simulink model "S5_MPC_Lab"  (R2025b)
settings: Solver=VariableStepAuto  StartTime=0.0  StopTime=200  FixedStep=0.5  MaxStep=0.05  RelTol=1e-3  AbsTol=1e-3
undefined symbols (not defined in the file or in its folder): g, gamma, mpc_Ts, q_in_step, T_water
libraries: nesl_utility x5, SimscapeFluids_lib x5, fl_lib x3, mpclib x1
settings Model: PacingRate=3.966100  Creator=emanu  LastModifiedBy=leffe
settings SolverCC: AutoScaleAbsTol=off  AlgebraicLoopSolver=TrustRegion  MaxZcPerStep=1.0
settings OptimizationCC: ReuseModelBlockBuffer=off
settings DebuggingCC: AlgebraicLoopMsg=none  UnconnectedInputMsg=warning  UnconnectedOutputMsg=warning  UnconnectedLineMsg=warning  SymbolicDimsDataTypeCodeGenerationDiagnostic=none
settings ModelReferenceCC: EnableRefExpFcnMdlSchedulingChecks=on
settings SFSimCC: CustomCodeUndefinedFunction=UseInterfaceOnly
settings RTWCC: GPUComputeCapability=3.5  DLArmComputeVersion=19.05
settings SimscapeCC: SimscapeLogDataHistory=10000.0

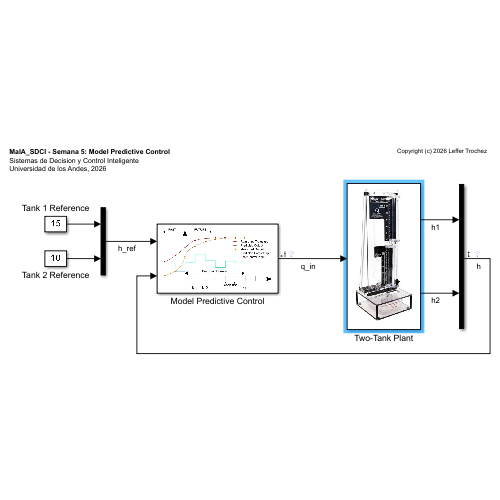
[thumbnail: Simulink's stored preview of the top-level diagram]
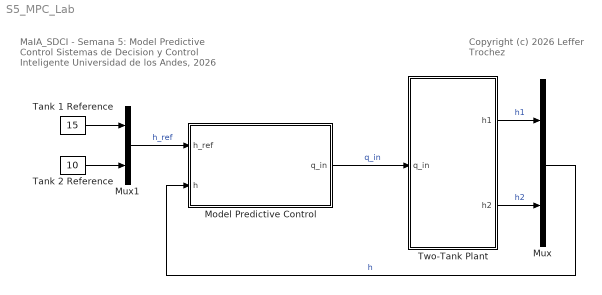
== system S5_MPC_Lab ==
  note: MaIA_SDCI - Semana 5: Model Predictive Control
      | Sistemas de Decision y Control Inteligente
      | Universidad de los Andes, 2026
  note: Copyright (c) 2026 Leffer Trochez
  Model Predictive Control : Subsystem
      mask Display: image('MPC.webp', [0,0,0,0,90,90]);
  Mux : Mux  Inputs=2
  Mux1 : Mux  Inputs=2
  Tank 1 Reference : Constant  Value=15
  Tank 2 Reference : Constant  Value=10
  Two-Tank Plant : Subsystem
      mask Display: image('Plant.jpeg');
  wires:
  Model Predictive Control/1(q_in) -> Two-Tank Plant/1(q_in)  "q_in"
  Two-Tank Plant/1(h1) -> Mux/1  "h1"
  Two-Tank Plant/2(h2) -> Mux/2  "h2"
  Mux/1 -> Model Predictive Control/2(h)  "h"
  Mux1/1 -> Model Predictive Control/1(h_ref)  "h_ref"
  Tank 1 Reference/1 -> Mux1/1
  Tank 2 Reference/1 -> Mux1/2

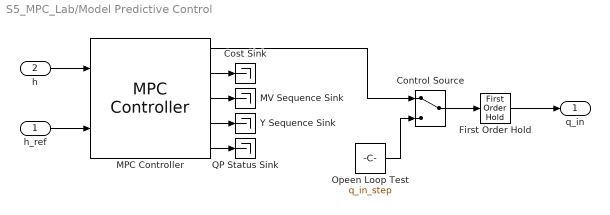
== system S5_MPC_Lab/Model Predictive Control ==
  h_ref : Inport
  h : Inport  Port=2
  " First Order Hold " : FirstOrderHold  ErrorTolerance=inf
  " MPC Controller " : mpclib/MPC Controller  SCDEnableBlockLinearizationSpecification=on  mpcobj=mpcController  is_multiple=0  enable_value=0  return_u0=off  updateMPCinCallerWorkspace=on  md_inport=off  mv_inport=off  uref_inport=off  return_cost=on  return_mvseq=on  return_qpstatus=on  return_xseq=off  return_state=off  return_ovseq=on  state_inport=off  umin_inport=off  umax_inport=off  ymin_inport=off  ymax_inport=off  cc_inport=off  ywt_inport=off  uwt_inport=off  duwt_inport=off  rhoeps_inport=off  pm_inport=off  MaximumP=10  HorizonChoice=FixedHorizon  n_ts=0.5  n_p=40  n_mv=1  n_md=0  n_ud=0  n_mo=2  n_uo=0  BlockDataType=double  SampleTimeInherited=off  switch_inport=off
  Control Source : ManualSwitch
  Cost Sink : Terminator
  MV Sequence Sink : Terminator
  Opeen Loop Test : Constant  Value=q_in_step  SampleTime=mpc_Ts
  QP Status Sink : Terminator
  Y Sequence Sink : Terminator
  q_in : Outport
  wires:
  h_ref/1 -> " MPC Controller "/2
  h/1 -> " MPC Controller "/1
  " First Order Hold "/1 -> q_in/1
  " MPC Controller "/1 -> Control Source/1
  Control Source/1 -> " First Order Hold "/1
  Opeen Loop Test/1 -> Control Source/2
  " MPC Controller "/2 -> Cost Sink/1
  " MPC Controller "/3 -> MV Sequence Sink/1
  " MPC Controller "/4 -> Y Sequence Sink/1
  " MPC Controller "/5 -> QP Status Sink/1

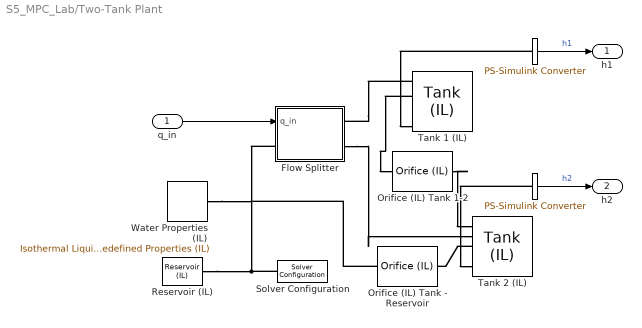
== system S5_MPC_Lab/Two-Tank Plant ==
  q_in : Inport
  " " : nesl_utility/PS-Simulink Converter  PhysicalDomain=network_engine_domain  SubClassName=ps_output  LeftPortType=input  RightPortType=output  PseudoPeriodic=off  Frequencies=[]  VectorFormat=inherit  Unit=cm  AffineConversion=off
  "  " : nesl_utility/PS-Simulink Converter  PhysicalDomain=network_engine_domain  SubClassName=ps_output  LeftPortType=input  RightPortType=output  PseudoPeriodic=off  Frequencies=[]  VectorFormat=inherit  Unit=cm  AffineConversion=off
  " Orifice (IL) Tank - Reservoir" : SimscapeFluids_lib/Isothermal Liquid/Valves & Orifices/Orifices/Orifice (IL)  orifice_type=foundation.enum.constant_variable.constant  constant_orifice_spec=fluids.isothermal_liquid.valves_orifices.orifices.enum.constant_orifice_spec.area  variable_orifice_spec=fluids.isothermal_liquid.valves_orifices.orifices.enum.orifice_spec.linear  orifice_area_constant=A_out cm^2  p_diff_TLU_constant=[-4, -3, -2, -1, -.5, 0, .5, 1, 2, 3, 4] MPa  vol_flow_TLU_constant=[-2.44, -2.12, -1.68, -1.22, -.84, 0, .85, 1.21, 1.7, 2.09, 2.41] .* 1e-3 m^3/s  S_min=0 m  del_S=5e-3 m  open_orientation=fluids.isothermal_liquid.valves_orifices.orifices.enum.orifice_orientation.positive  area_max=1e-4 m^2  area_leak=1e-10 m^2  S_TLU=[0, .002, .004, .007, .017] m  orifice_area_TLU=[1e-09, 2.0352e-07, 4.0736e-05, .00011438, .00034356] m^2  area=inf cm^2  Cd=0.64  Re_c=150  smoothing_factor=0.01  pressure_recovery=false  S_vol_flow_TLU=[0, .002, .004, .007, .017] m  p_diff_TLU=[.3, .5, .7] MPa  vol_flow_TLU=1e-3 * [1.7e-05, 2e-05, 2.6e-05; .0035, .0045, .0053; .7, .9, 1.06; 1.96, 2.5, 3; 6, 7.7, 9.13] m^3/s
      settings: InternalSimscapePortConfiguration="{\"Bottom\":[],\"Left\":[{\"id\":\"A\",\"label\":\"A\",\"type\":\"foundation.isothermal_liquid.isothermal_liquid\"}],\"Right\":[{\"id\":\"B\",\"label\":\"B\",\"type\":\"foundation.isothermal_liquid.isothermal_liquid\"}],\"Top\":[]}"
  " Orifice (IL) Tank 1-2" : SimscapeFluids_lib/Isothermal Liquid/Valves & Orifices/Orifices/Orifice (IL)  orifice_type=foundation.enum.constant_variable.constant  constant_orifice_spec=fluids.isothermal_liquid.valves_orifices.orifices.enum.constant_orifice_spec.area  variable_orifice_spec=fluids.isothermal_liquid.valves_orifices.orifices.enum.orifice_spec.linear  orifice_area_constant=A_12 cm^2  p_diff_TLU_constant=[-4, -3, -2, -1, -.5, 0, .5, 1, 2, 3, 4] MPa  vol_flow_TLU_constant=[-2.44, -2.12, -1.68, -1.22, -.84, 0, .85, 1.21, 1.7, 2.09, 2.41] .* 1e-3 m^3/s  S_min=0 m  del_S=5e-3 m  open_orientation=fluids.isothermal_liquid.valves_orifices.orifices.enum.orifice_orientation.positive  area_max=1e-4 m^2  area_leak=1e-10 m^2  S_TLU=[0, .002, .004, .007, .017] m  orifice_area_TLU=[1e-09, 2.0352e-07, 4.0736e-05, .00011438, .00034356] m^2  area=inf cm^2  Cd=0.64  Re_c=150  smoothing_factor=0.01  pressure_recovery=false  S_vol_flow_TLU=[0, .002, .004, .007, .017] m  p_diff_TLU=[.3, .5, .7] MPa  vol_flow_TLU=1e-3 * [1.7e-05, 2e-05, 2.6e-05; .0035, .0045, .0053; .7, .9, 1.06; 1.96, 2.5, 3; 6, 7.7, 9.13] m^3/s
      settings: InternalSimscapePortConfiguration="{\"Bottom\":[],\"Left\":[{\"id\":\"A\",\"label\":\"A\",\"type\":\"foundation.isothermal_liquid.isothermal_liquid\"}],\"Right\":[{\"id\":\"B\",\"label\":\"B\",\"type\":\"foundation.isothermal_liquid.isothermal_liquid\"}],\"Top\":[]}"
  Flow Splitter : Subsystem
      mask Display: image('$imagefile'); % Use "Edit Image" on toolstrip to change.
  Reservoir (IL) : fl_lib/Isothermal Liquid/Elements/Reservoir (IL)  reservoir_type=foundation.enum.constant_controlled.constant  pressure_spec=foundation.enum.pressure_spec.specified  reservoir_pressure=p_env atm
  Solver Configuration : nesl_utility/Solver Configuration  PhysicalDomain=network_engine_domain  SubClassName=solver  LeftPortType=input  RightPortType=generic  Tones=[]  Harmonics=[]  SimulateNoise=off  Profile=off  UseLocalSampling=off  EnableSwitchedLinearOptims=on  FrequencyDomain=off  UseCCode=off  RelTol=0.001  AbsTol=1e-06  MinStep=1e-09  ToWorkspace=off  RevertToSquareIcSolve=off  NumHomotopyIterations=100  PhasorMode=off  PhasorModeNumHarmonics=1  ConsistencySolver=NEWTON_XTOL_AFTER_FTOL  IndexReductionMethod=DerivativeReplacement  DoDC=off  ResidualTolerance=1e-09  ConsistencyTolSource=GLOBAL  ConsistencyAbsTol=0.001  ConsistencyRelTol=0.001  ConsistencyTolFactor=0.001  UseLocalSolver=off  LocalSolverChoice=NE_BACKWARD_EULER_ADVANCER  ResolveIndetEquations=on  FunctionEvalNumThread=1  LocalSolverSampleTime=0.001  DoFixedCost=on  MaxNonlinIter=3  MaxModeIter=2  ComputeImpulses=off  ImpulseIterations=2  LinearAlgebra=auto  LinearAlgebraNumThread=0  EquationFormulation=NE_TIME_EF  DelaysMemoryBudget=1024  AutomaticFiltering=on  FilteringTimeConstant=0.001  PartitionStorageMethod=AS_NEEDED  PartitionMemoryBudget=1024  PartitionMethod=ROBUST  MultibodyUseLocalSolver=off  MultibodyLocalSolverChoice=ODE1  MultibodyLocalSolverSampleTime=0.001
  Tank 1 (IL) : SimscapeFluids_lib/Isothermal Liquid/Tanks & Accumulators/Tank (IL)  num_inlet=fluids.isothermal_liquid.tanks_accumulators.enum.NumInlet.Two  pressure_spec=foundation.enum.pressure_spec.specified  tank_pressure=p_env atm  volume_spec=fluids.isothermal_liquid.tanks_accumulators.enum.TankVolumeSpec.Constant  tank_area=A_tank cm^2  level_TLU=[0, 3, 5] m  volume_TLU=[0, 4, 6] m^3  inlet_height_A=0.1 m  inlet_area_A=0.01 m^2  inlet_height_AB=h_ports_T1 cm  inlet_area_AB=A_ports_T1 cm^2  inlet_height_ABC=[.1, .1, .1] m  inlet_area_ABC=[.01, .01, .01] m^2  inlet_height_ABCD=0.1 * ones(1, 4) m  inlet_area_ABCD=0.01 * ones(1, 4) m^2  inlet_height_ABCDE=0.1 * ones(1, 5) m  inlet_area_ABCDE=0.01 * ones(1, 5) m^2  inlet_height_ABCDEF=0.1 * ones(1, 6) m  inlet_area_ABCDEF=0.01 * ones(1, 6) m^2  level_check=simscape.enum.assert.action.none  capacity_check=simscape.enum.assert.action.warn  max_capacity=V_max cm^3  g=g m/s^2  level_specify=on  level_priority=High  level=h1_0 cm  level_nominal_specify=off  level_nominal_value=1  level_nominal_unit=m  volume_specify=off  volume_priority=None  volume=0 cm^3  volume_nominal_specify=off  volume_nominal_value=1  volume_nominal_unit=m^3  mass_specify=off  mass_priority=None  mass=0 kg  mass_nominal_specify=off  mass_nominal_value=1  mass_nominal_unit=kg
      settings: InternalSimscapePortConfiguration="{\"Bottom\":[],\"Left\":[{\"id\":\"A\",\"label\":\"A\",\"type\":\"foundation.isothermal_liquid.isothermal_liquid\"},{\"id\":\"B\",\"label\":\"B\",\"type\":\"foundation.isothermal_liquid.isothermal_liquid\"}],\"Right\":[],\"Top\":[{\"id\":\"V\",\"label\":\"V\",\"type\":\"output\"},{\"id\":\"L\",\"label\":\"L\",\"type\":\"output\"}]}"
  Tank 2 (IL) : SimscapeFluids_lib/Isothermal Liquid/Tanks & Accumulators/Tank (IL)  num_inlet=fluids.isothermal_liquid.tanks_accumulators.enum.NumInlet.Three  pressure_spec=foundation.enum.pressure_spec.specified  tank_pressure=p_env atm  volume_spec=fluids.isothermal_liquid.tanks_accumulators.enum.TankVolumeSpec.Constant  tank_area=A_tank cm^2  level_TLU=[0, 3, 5] m  volume_TLU=[0, 4, 6] m^3  inlet_height_A=0.1 m  inlet_area_A=0.01 m^2  inlet_height_AB=[.1, .1] m  inlet_area_AB=[.01, .01] m^2  inlet_height_ABC=h_ports_T2 cm  inlet_area_ABC=A_ports_T2 cm^2  inlet_height_ABCD=0.1 * ones(1, 4) m  inlet_area_ABCD=0.01 * ones(1, 4) m^2  inlet_height_ABCDE=0.1 * ones(1, 5) m  inlet_area_ABCDE=0.01 * ones(1, 5) m^2  inlet_height_ABCDEF=0.1 * ones(1, 6) m  inlet_area_ABCDEF=0.01 * ones(1, 6) m^2  level_check=simscape.enum.assert.action.none  capacity_check=simscape.enum.assert.action.warn  max_capacity=V_max cm^3  g=g m/s^2  level_specify=on  level_priority=High  level=h2_0 cm  level_nominal_specify=off  level_nominal_value=1  level_nominal_unit=m  volume_specify=off  volume_priority=None  volume=0 m^3  volume_nominal_specify=off  volume_nominal_value=1  volume_nominal_unit=m^3  mass_specify=off  mass_priority=None  mass=0 kg  mass_nominal_specify=off  mass_nominal_value=1  mass_nominal_unit=kg
      settings: InternalSimscapePortConfiguration="{\"Bottom\":[],\"Left\":[{\"id\":\"A\",\"label\":\"A\",\"type\":\"foundation.isothermal_liquid.isothermal_liquid\"},{\"id\":\"B\",\"label\":\"B\",\"type\":\"foundation.isothermal_liquid.isothermal_liquid\"},{\"id\":\"C\",\"label\":\"C\",\"type\":\"foundation.isothermal_liquid.isothermal_liquid\"}],\"Right\":[],\"Top\":[{\"id\":\"V\",\"label\":\"V\",\"type\":\"output\"},{\"id\":\"L\",\"label\":\"L\",\"type\":\"output\"}]}"
  Water Properties (IL) : SimscapeFluids_lib/Isothermal Liquid/Utilities/Isothermal Liquid Predefined Properties (IL)  fluid_list=fluids.isothermal_liquid.utilities.enum.isothermal_liquid_fluid_list.water  concentration_param_EG=fluids.isothermal_liquid.utilities.enum.isothermal_liquid_concentration.volume_fraction  concentration_param_PG=fluids.isothermal_liquid.utilities.enum.isothermal_liquid_concentration.volume_fraction  c_mass_SW=3.5e-3  c_mass_EG=0.1  c_mass_PG=0.1  c_mass_GL=0.1  c_vol_EG=0.1  c_vol_PG=0.1  beta_L_atm_EG=2.1791 GPa  beta_L_atm_PG=2.1791 GPa  beta_L_atm_GL=2.1791 GPa  p_min_EG=0.01 MPa  p_min_PG=0.01 MPa  p_min_GL=0.01 MPa  T=T_water K  derate_coeff=1  p_atm=0.101325 MPa  properties_range_check=simscape.enum.assert.action.error  air_fraction=0.005  polytropic_index=1.0  rho_g_atm=1.225 kg/m^3  air_dissolution_model=simscape.enum.onoff.off  p_crit=3 MPa
      settings: InternalSimscapePortConfiguration="{\"Bottom\":[],\"Left\":[],\"Right\":[{\"id\":\"A\",\"label\":\"\",\"type\":\"foundation.isothermal_liquid.isothermal_liquid\"}],\"Top\":[]}"
  h1 : Outport
  h2 : Outport  Port=2
  wires:
  " "/1 -> h1/1  "h1"
  "  "/1 -> h2/1  "h2"
  q_in/1 -> Flow Splitter/1(q_in)
  connections:
  Flow Splitter/RConn2 -- Tank 2 (IL)/LConn2
  Reservoir (IL)/LConn1 -- " Orifice (IL) Tank - Reservoir"/RConn1 -- Flow Splitter/LConn1 -- Water Properties (IL)/RConn1 -- Solver Configuration/RConn1
  "  "/LConn1 -- Tank 2 (IL)/LConn5
  " "/LConn1 -- Tank 1 (IL)/LConn4
  Tank 1 (IL)/LConn1 -- Flow Splitter/RConn1
  Tank 1 (IL)/LConn2 -- " Orifice (IL) Tank 1-2"/LConn1
  " Orifice (IL) Tank 1-2"/RConn1 -- Tank 2 (IL)/LConn1
  Tank 2 (IL)/LConn3 -- " Orifice (IL) Tank - Reservoir"/LConn1

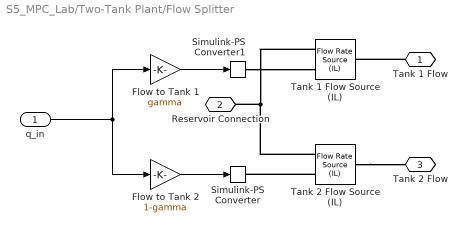
== system S5_MPC_Lab/Two-Tank Plant/Flow Splitter ==
  q_in : Inport
  Flow to Tank 1 : Gain  Gain=gamma
  Flow to Tank 2 : Gain  Gain=1-gamma
  Simulink-PS Converter : nesl_utility/Simulink-PS Converter  PhysicalDomain=network_engine_domain  SubClassName=ps_input  LeftPortType=input  RightPortType=output  PseudoPeriodic=off  Frequencies=[]  NoiseDistribution=none  NoiseParameters=[]  Unit=cm^3/s  AffineConversion=off  FilteringAndDerivatives=provide  SimscapeFilterOrder=1  InputFilterTimeConstant=0.001  UdotUserProvided=0
  Simulink-PS Converter1 : nesl_utility/Simulink-PS Converter  PhysicalDomain=network_engine_domain  SubClassName=ps_input  LeftPortType=input  RightPortType=output  PseudoPeriodic=off  Frequencies=[]  NoiseDistribution=none  NoiseParameters=[]  Unit=cm^3/s  AffineConversion=off  FilteringAndDerivatives=provide  SimscapeFilterOrder=1  InputFilterTimeConstant=0.001  UdotUserProvided=0
  Tank 1 Flow Source (IL) : fl_lib/Isothermal Liquid/Sources/Flow Rate Source (IL)  source_type=foundation.enum.constant_controlled.controlled  flow_type=foundation.enum.mass_volumetric_flow.volumetric  mass_flow=0 kg/s  volumetric_flow=27*0.4 gpm
      settings: InternalSimscapePortConfiguration="{\"Bottom\":[],\"Left\":[{\"id\":\"A\",\"label\":\"A\",\"type\":\"foundation.isothermal_liquid.isothermal_liquid\"},{\"id\":\"V\",\"label\":\"V\",\"type\":\"input\"}],\"Right\":[{\"id\":\"B\",\"label\":\"B\",\"type\":\"foundation.isothermal_liquid.isothermal_liquid\"}],\"Top\":[]}"
  Tank 2 Flow Source (IL) : fl_lib/Isothermal Liquid/Sources/Flow Rate Source (IL)  source_type=foundation.enum.constant_controlled.controlled  flow_type=foundation.enum.mass_volumetric_flow.volumetric  mass_flow=0 kg/s  volumetric_flow=27*0.6 gpm
      settings: InternalSimscapePortConfiguration="{\"Bottom\":[],\"Left\":[{\"id\":\"A\",\"label\":\"A\",\"type\":\"foundation.isothermal_liquid.isothermal_liquid\"},{\"id\":\"V\",\"label\":\"V\",\"type\":\"input\"}],\"Right\":[{\"id\":\"B\",\"label\":\"B\",\"type\":\"foundation.isothermal_liquid.isothermal_liquid\"}],\"Top\":[]}"
  Tank 1 Flow : PMIOPort  Side=Right
  Reservoir Connection : PMIOPort  Port=2  Side=Left
  Tank 2 Flow : PMIOPort  Port=3  Side=Right
  wires:
  Flow to Tank 1/1 -> Simulink-PS Converter1/1
  Flow to Tank 2/1 -> Simulink-PS Converter/1
  q_in/1 -> Flow to Tank 2/1, Flow to Tank 1/1
  connections:
  Tank 2 Flow Source (IL)/LConn1 -- Tank 1 Flow Source (IL)/LConn1 -- Reservoir Connection/RConn1
  Tank 2 Flow Source (IL)/RConn1 -- Tank 2 Flow/RConn1
  Tank 1 Flow/RConn1 -- Tank 1 Flow Source (IL)/RConn1
  Simulink-PS Converter1/RConn1 -- Tank 1 Flow Source (IL)/LConn2
  Tank 2 Flow Source (IL)/LConn2 -- Simulink-PS Converter/RConn1
